simulink model "PV_Array_Subsystem"  (R2025a)
settings: Solver=ode45  StartTime=0.0  StopTime=86400  MaxStep=1e-4  MinStep=1e-8  RelTol=1e-5  AbsTol=1e-8
settings Model: Creator=denis  LastModifiedBy=denis

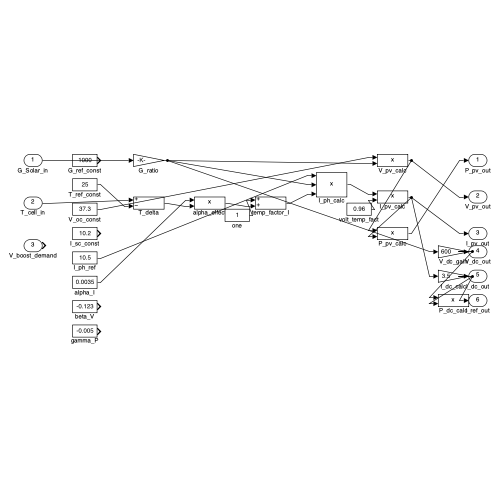
[thumbnail: Simulink's stored preview of the top-level diagram]
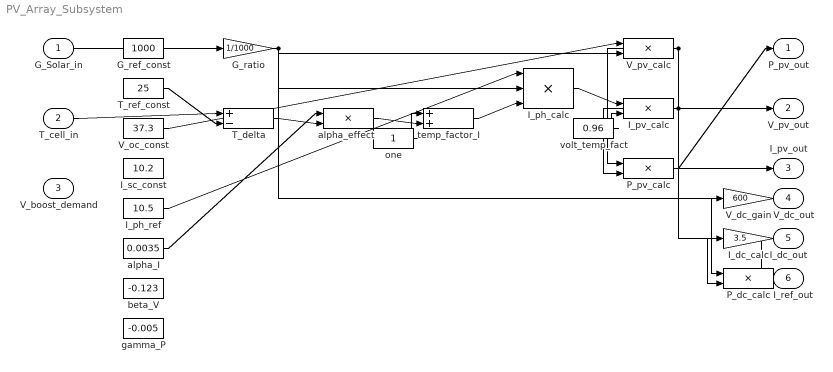
== system PV_Array_Subsystem ==
  G_Solar_in : Inport
  T_cell_in : Inport  Port=2
  V_boost_demand : Inport  Port=3
  G_ratio : Gain  Gain=1/1000
  G_ref_const : Constant  Value=1000
  I_dc_calc : Gain  Gain=3.5
  I_ph_calc : Product  Inputs=3
  I_ph_ref : Constant  Value=10.5
  I_pv_calc : Product
  I_sc_const : Constant  Value=10.2
  P_dc_calc : Product
  P_pv_calc : Product
  T_delta : Sum  Inputs=+-
  T_ref_const : Constant  Value=25
  V_dc_gain : Gain  Gain=600
  V_oc_const : Constant  Value=37.3
  V_pv_calc : Product
  alpha_I : Constant  Value=0.0035
  alpha_effect : Product
  beta_V : Constant  Value=-0.123
  gamma_P : Constant  Value=-0.005
  one : Constant
  temp_factor_I : Sum
  volt_temp_fact : Constant  Value=0.96
  P_pv_out : Outport
  V_pv_out : Outport  Port=2
  I_pv_out : Outport  Port=3
  V_dc_out : Outport  Port=4
  I_dc_out : Outport  Port=5
  I_ref_out : Outport  Port=6
  wires:
  G_Solar_in/1 -> G_ratio/1
  T_cell_in/1 -> T_delta/1
  T_ref_const/1 -> T_delta/2
  alpha_I/1 -> alpha_effect/1
  T_delta/1 -> alpha_effect/2
  one/1 -> temp_factor_I/1
  alpha_effect/1 -> temp_factor_I/2
  I_ph_ref/1 -> I_ph_calc/1
  G_ratio/1 -> I_ph_calc/2, V_pv_calc/2, V_dc_gain/1
  temp_factor_I/1 -> I_ph_calc/3
  V_oc_const/1 -> V_pv_calc/1
  I_ph_calc/1 -> I_pv_calc/1
  volt_temp_fact/1 -> I_pv_calc/2
  V_pv_calc/1 -> P_pv_calc/1, V_pv_out/1
  I_pv_calc/1 -> P_pv_calc/2, I_dc_calc/1, I_pv_out/1
  V_dc_gain/1 -> P_dc_calc/1, V_dc_out/1
  I_dc_calc/1 -> P_dc_calc/2, I_dc_out/1, I_ref_out/1
  P_pv_calc/1 -> P_pv_out/1
